simulink model "enr312_dc_motor"  (R2026a)
settings: Solver=ode45  StopTime=Tend  MaxStep=1e-3  RelTol=1e-8  AbsTol=1e-10
model workspace (MAT data in the model file):
  J = 1e-06
  Kd = 0
  Ke = 0.00568713663315
  Ki = 1
  Kp = 0.05
  Kt = 0.00568713663315
  L = 0.0005
  N = 100
  R = 1.6
  Tend = 5
  Tf = 0.01
  Ts = 0.01
  b = 2.41369575255e-06
  closedLoop = 1
  dist = 0
  eta = 1
  ffGain = 0.0666666666667
  loopSel = 1
  qInt = 0.0692307692308
  setpoint = 100
  tDist = 3
  tStep = 0.2
  uMax = 12
libraries: slpidlib x1, simulink x1
settings Model: Creator=odyssix  LastModifiedBy=odyssix

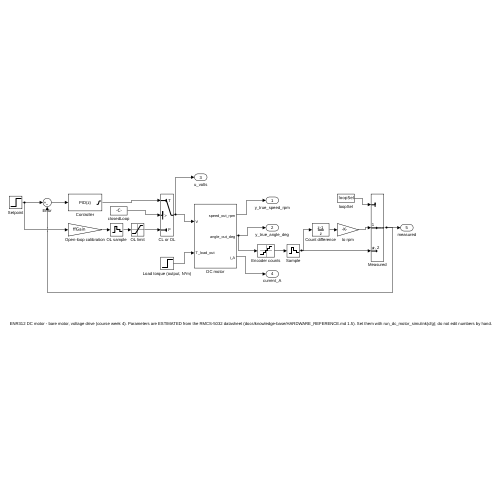
[thumbnail: Simulink's stored preview of the top-level diagram]
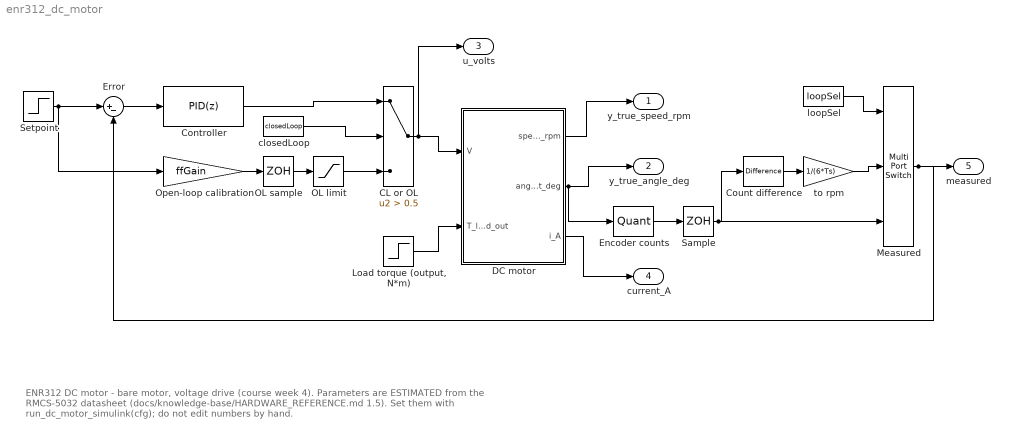
== system enr312_dc_motor ==
  note: ENR312 DC motor - bare motor, voltage drive (course week 4). Parameters are ESTIMATED from the RMCS-5032 datasheet (docs/knowledge-base/HARDWARE_REFERENCE.md 1.5). Set them with run_dc_motor_simulink(cfg); do not edit numbers by hand.
  CL or OL : Switch  Criteria=u2 > Threshold  Threshold=0.5  SaturateOnIntegerOverflow=off  InputSameDT=off
  Controller : slpidlib/PID Controller  Controller=PID  Form=Parallel  TimeDomain=Discrete-time  UseExternalTs=off  SampleTime=Ts  IntegratorMethod=Backward Euler  FilterMethod=Backward Euler  ControllerParametersSource=internal  P=Kp  I=Ki  UseKiTs=off  D=Kd  UseExternalDerivativeSource=off  N=1/Tf  UseFilter=on  TunerSelectOption=Transfer Function Based (PID Tuner App)  InitialConditionSource=internal  InitialConditionForIntegrator=0  InitialConditionForFilter=0  DifferentiatorICPrevScaledInput=0  ExternalReset=none  TrackingMode=off  Kt=1  LimitOutput=on  SatLimitsSource=internal  UpperSaturationLimit=uMax  LowerSaturationLimit=-uMax  LinearizeAsGain=off  AntiWindupMode=clamping  Kb=1  LimitIntegrator=off  UpperIntegratorSaturationLimit=inf  LowerIntegratorSaturationLimit=-inf  POutMin=[]  POutMax=[]  IOutMin=[]  IOutMax=[]  DOutMin=[]  DOutMax=[]  NOutMin=[]  NOutMax=[]  SumOutMin=[]  SumOutMax=[]  SaturationOutMin=[]  SaturationOutMax=[]  PParamMin=[]  PParamMax=[]  IParamMin=[]  IParamMax=[]  DParamMin=[]  DParamMax=[]  NParamMin=[]  NParamMax=[]  KbParamMin=[]  KbParamMax=[]  KtParamMin=[]  KtParamMax=[]  KbOutMin=[]  KbOutMax=[]  KtOutMin=[]  KtOutMax=[]  IntegratorOutMin=[]  IntegratorOutMax=[]  FilterOutMin=[]  FilterOutMax=[]  SumI1OutMin=[]  SumI1OutMax=[]  SumI2OutMin=[]  SumI2OutMax=[]  SumI3OutMin=[]  SumI3OutMax=[]  SumI4OutMin=[]  SumI4OutMax=[]  SumDOutMin=[]  SumDOutMax=[]  DifferentiatorOutMin=[]  DifferentiatorOutMax=[]  FilterDiffOutCoefMin=[]  FilterDiffOutCoefMax=[]  ReciprocalOutMin=[]  ReciprocalOutMax=[]  SumDenOutMin=[]  SumDenOutMax=[]  SumNumOutMin=[]  SumNumOutMax=[]  DivideOutMin=[]  DivideOutMax=[]  UdiffTsProdOutMin=[]  UdiffTsProdOutMax=[]  NTsProdOutMin=[]  NTsProdOutMax=[]  UintegralTsProdOutMin=[]  UintegralTsProdOutMax=[]  UngainTsProdOutMin=[]  UngainTsProdOutMax=[]  ClampingZeroOutDataTypeStr=Inherit: Inherit via back propagation  ClampingZeroOutMin=[]  ClampingZeroOutMax=[]  FilterDenConstantOutDataTypeStr=Inherit: Inherit via back propagation  FilterDenConstantOutMin=[]  FilterDenConstantOutMax=[]  PCopyOutDataTypeStr=Inherit: Inherit via back propagation  PCopyOutMin=[]  PCopyOutMax=[]  NCopyOutDataTypeStr=Inherit: Inherit via back propagation  NCopyOutMin=[]  NCopyOutMax=[]  IntegratorContinuousStateAttributes=''  IntegratorStateMustResolveToSignalObject=off  IntegratorRTWStateStorageClass=Auto  FilterContinuousStateAttributes=''  FilterStateMustResolveToSignalObject=off  FilterRTWStateStorageClass=Auto  ParallelPVariant=InternalParameters  IdealPVariant=Disabled  IVariant=InternalParameters  DVariant=InternalParameters  IntegratorVariant=Discrete  SatVariant=Enabled  AWVariant=DiscClampingParallel  PCopyVariant=Disabled  TRVariant=Disabled  FdbkBlocksVariant=Feedback  IdealPFdbkVariant=Passthrough  SatFdbkVariant=Passthrough  DerivativeFilterVariant=BackwardEulerFilter  NVariant=InternalParameters  NCopyVariant=InternalParameters  FilterICVariant=InternalICsFilter  IntegratorICVariant=InternalICs  ExternalResetVariant=Disabled  TRSumVariant=Passthrough  SumFdbkVariant=Enabled  SumVariant=Sum_PID  TsampFilterVariant=InternalTs  TsampNgainVariant=Passthrough  TsampIntegralVariant=Disabled_SignalSpec  ExternalSaturationOutDataTypeStr=Inherit: Same as second input  DerivativeSourceVariant=ErrorSignal  PreIntVariant=InternalPreInt
      settings: LibrarySourceBlock=simulink/Discrete/Discrete PID Controller
  Count difference : simulink/Discrete/Difference  ICPrevInput=0.0  OutMin=[]  OutMax=[]  OutDataType=fixdt(1, 16)  OutScaling=2^-10  DoSatur=off
  DC motor : Subsystem
  Encoder counts : Quantizer  QuantizationInterval=qInt
  Error : Sum  Inputs=|+-
  "Load torque (output, N*m)" : Step  Time=tDist  FinalValue=dist  SampleTime=0
  Measured : MultiPortSwitch  Inputs=2  SaturateOnIntegerOverflow=off  InputSameDT=off
  OL limit : Saturate  UpperLimit=uMax  LowerLimit=-uMax
  OL sample : ZeroOrderHold  SampleTime=Ts
  Open-loop calibration : Gain  Gain=ffGain
  Sample : ZeroOrderHold  SampleTime=Ts
  Setpoint : Step  Time=tStep  FinalValue=setpoint  SampleTime=0
  closedLoop : Constant  Value=closedLoop
  loopSel : Constant  Value=loopSel
  to rpm : Gain  Gain=1/(6*Ts)
  y_true_speed_rpm : Outport
  y_true_angle_deg : Outport  Port=2
  u_volts : Outport  Port=3
  current_A : Outport  Port=4
  measured : Outport  Port=5
  wires:
  Setpoint/1 -> Error/1, Open-loop calibration/1
  Error/1 -> Controller/1
  Controller/1 -> CL or OL/1
  closedLoop/1 -> CL or OL/2
  Open-loop calibration/1 -> OL sample/1
  OL sample/1 -> OL limit/1
  OL limit/1 -> CL or OL/3
  CL or OL/1 -> DC motor/1(V), u_volts/1
  "Load torque (output, N*m)"/1 -> DC motor/2(T_load_out)
  DC motor/1(speed_out_rpm) -> y_true_speed_rpm/1
  DC motor/2(angle_out_deg) -> y_true_angle_deg/1, Encoder counts/1
  DC motor/3(i_A) -> current_A/1
  Encoder counts/1 -> Sample/1
  Sample/1 -> Count difference/1, Measured/3
  Count difference/1 -> to rpm/1
  loopSel/1 -> Measured/1
  to rpm/1 -> Measured/2
  Measured/1 -> Error/2, measured/1

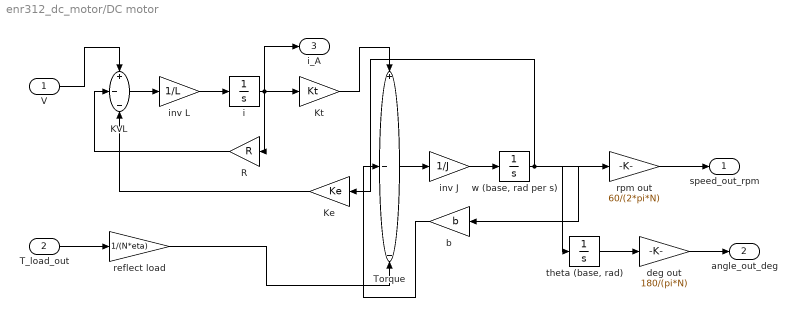
== system enr312_dc_motor/DC motor ==
  V : Inport
  T_load_out : Inport  Port=2
  KVL : Sum  Inputs=+--
  Ke : Gain  Gain=Ke
  Kt : Gain  Gain=Kt
  R : Gain  Gain=R
  Torque : Sum  Inputs=+--
  b : Gain  Gain=b
  deg out : Gain  Gain=180/(pi*N)
  i : Integrator
  inv J : Gain  Gain=1/J
  inv L : Gain  Gain=1/L
  reflect load : Gain  Gain=1/(N*eta)
  rpm out : Gain  Gain=60/(2*pi*N)
  "theta (base, rad)" : Integrator
  "w (base, rad per s)" : Integrator
  speed_out_rpm : Outport
  angle_out_deg : Outport  Port=2
  i_A : Outport  Port=3
  wires:
  V/1 -> KVL/1
  KVL/1 -> inv L/1
  inv L/1 -> i/1
  i/1 -> Kt/1, R/1, i_A/1
  R/1 -> KVL/2
  Kt/1 -> Torque/1
  Torque/1 -> inv J/1
  inv J/1 -> "w (base, rad per s)"/1
  "w (base, rad per s)"/1 -> b/1, Ke/1, "theta (base, rad)"/1, rpm out/1
  b/1 -> Torque/2
  Ke/1 -> KVL/3
  T_load_out/1 -> reflect load/1
  reflect load/1 -> Torque/3
  rpm out/1 -> speed_out_rpm/1
  "theta (base, rad)"/1 -> deg out/1
  deg out/1 -> angle_out_deg/1
